simulink model "gnc_model_flightgear"  (R2026a)
settings: Solver=VariableStepAuto  StopTime=500
values from neighbouring files (symbols this model uses):
  B = [-0.25; -331.40]    [gnc_parameters.m]
  C = [-123.34, 0 ; 0, 1]    [gnc_parameters.m]
  D = [-13.51; 0]    [gnc_parameters.m]
  d2r = pi/180    (= 0.0174532925199)    [gnc_parameters.m]
  dT1 = 0.75    [gnc_parameters.m]
  dT2 = 0.25    [gnc_parameters.m]
  Elev_init = 10000    [gnc_parameters.m]
  Elev_target = 800    [gnc_parameters.m]
  Lat_init = 34.2329    [gnc_parameters.m]
  Lat_obs = 34.608485    [gnc_parameters.m]
  Lat_target = 34.6624    [gnc_parameters.m]
  Lon_init = -119.4573    [gnc_parameters.m]
  Lon_obs = -118.867712    [gnc_parameters.m]
  Lon_target = -118.7629    [gnc_parameters.m]
  m2f = 3.2811    [gnc_parameters.m]
  Vel = 3021.08    [gnc_parameters.m]
  yaw = yaw_init*d2r    [gnc_parameters.m]
undefined symbols (not defined in the file or in its folder): A, K, L
libraries: simulink x3, aerolibfltsims x2, slpidlib x1, aerolibanimutils x1
settings Model: Creator=natha  LastModifiedBy=natha

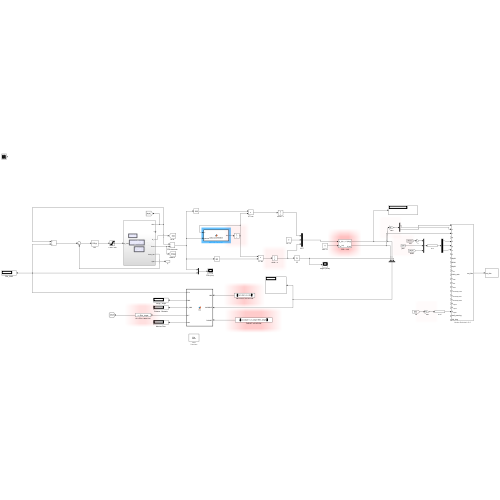
[thumbnail: Simulink's stored preview of the top-level diagram]
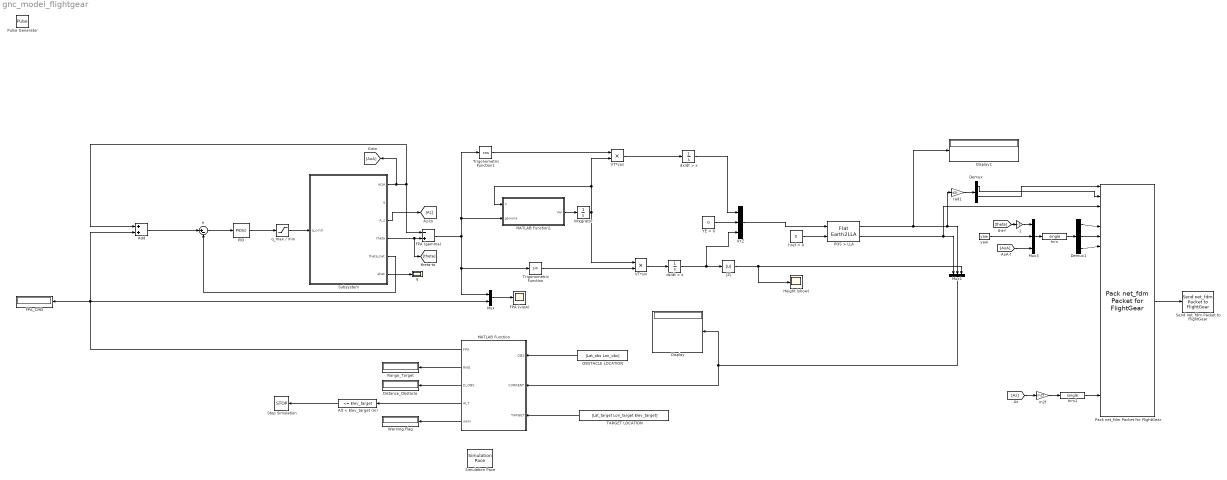
== system gnc_model_flightgear ==
  -1 : Gain  Gain=-1
  Add : Sum
  Alt < Elev_target (m) : simulink/Logic and Bit Operations/Compare To Constant  relop=<=  const=Elev_target  OutDataTypeStr=boolean
  Demux : Demux  Outputs=2
  Demux1 : Demux  Outputs=3
  Display : Display
  Display1 : Display
  Distance_Obstacle : Display
  FPA (gamma) : Sum  Inputs=-+
  FPA (view) : Scope
      settings: ActiveDisplayYMinimum=-0.063895204469408745  ActiveDisplayYMaximum=0.31656859228067386
  FPA_CMD : Display
  Height (show) : Scope
      settings: ActiveDisplayYMinimum=-1013.2400702404138  ActiveDisplayYMaximum=20440.633073900935  DataLoggingVariableName=ScopeData2
  Integrator : Integrator  InitialCondition=Vel
  MATLAB Function : MATLAB Function  TreatAsAtomicUnit=on
  MATLAB Function1 : MATLAB Function  TreatAsAtomicUnit=on
  Mux : Mux  Inputs=2
  Mux1 : Mux  Inputs=3
  Mux3 : Mux  Inputs=3
  OBSTACLE LOCATION : Constant  Value=[Lat_obs Lon_obs]
  "PID " : slpidlib/PID Controller  Controller=PID  Form=Parallel  TimeDomain=Continuous-time  UseExternalTs=off  SampleTime=-1  IntegratorMethod=Forward Euler  FilterMethod=Forward Euler  ControllerParametersSource=internal  P=-1  I=0  UseKiTs=off  D=0  UseExternalDerivativeSource=off  N=100  UseFilter=on  TunerSelectOption=Transfer Function Based (PID Tuner App)  InitialConditionSource=internal  InitialConditionForIntegrator=0  InitialConditionForFilter=0  DifferentiatorICPrevScaledInput=0  ExternalReset=none  TrackingMode=off  Kt=1  LimitOutput=off  SatLimitsSource=internal  UpperSaturationLimit=inf  LowerSaturationLimit=-inf  LinearizeAsGain=on  AntiWindupMode=none  Kb=1  LimitIntegrator=off  UpperIntegratorSaturationLimit=inf  LowerIntegratorSaturationLimit=-inf  POutMin=[]  POutMax=[]  IOutMin=[]  IOutMax=[]  DOutMin=[]  DOutMax=[]  NOutMin=[]  NOutMax=[]  SumOutMin=[]  SumOutMax=[]  SaturationOutMin=[]  SaturationOutMax=[]  PParamMin=[]  PParamMax=[]  IParamMin=[]  IParamMax=[]  DParamMin=[]  DParamMax=[]  NParamMin=[]  NParamMax=[]  KbParamMin=[]  KbParamMax=[]  KtParamMin=[]  KtParamMax=[]  KbOutMin=[]  KbOutMax=[]  KtOutMin=[]  KtOutMax=[]  IntegratorOutMin=[]  IntegratorOutMax=[]  FilterOutMin=[]  FilterOutMax=[]  SumI1OutMin=[]  SumI1OutMax=[]  SumI2OutMin=[]  SumI2OutMax=[]  SumI3OutMin=[]  SumI3OutMax=[]  SumI4OutMin=[]  SumI4OutMax=[]  SumDOutMin=[]  SumDOutMax=[]  DifferentiatorOutMin=[]  DifferentiatorOutMax=[]  FilterDiffOutCoefMin=[]  FilterDiffOutCoefMax=[]  ReciprocalOutMin=[]  ReciprocalOutMax=[]  SumDenOutMin=[]  SumDenOutMax=[]  SumNumOutMin=[]  SumNumOutMax=[]  DivideOutMin=[]  DivideOutMax=[]  UdiffTsProdOutMin=[]  UdiffTsProdOutMax=[]  NTsProdOutMin=[]  NTsProdOutMax=[]  UintegralTsProdOutMin=[]  UintegralTsProdOutMax=[]  UngainTsProdOutMin=[]  UngainTsProdOutMax=[]  ClampingZeroOutDataTypeStr=Inherit: Inherit via back propagation  ClampingZeroOutMin=[]  ClampingZeroOutMax=[]  FilterDenConstantOutDataTypeStr=Inherit: Inherit via back propagation  FilterDenConstantOutMin=[]  FilterDenConstantOutMax=[]  PCopyOutDataTypeStr=Inherit: Inherit via back propagation  PCopyOutMin=[]  PCopyOutMax=[]  NCopyOutDataTypeStr=Inherit: Inherit via back propagation  NCopyOutMin=[]  NCopyOutMax=[]  IntegratorContinuousStateAttributes=''  IntegratorStateMustResolveToSignalObject=off  IntegratorRTWStateStorageClass=Auto  FilterContinuousStateAttributes=''  FilterStateMustResolveToSignalObject=off  FilterRTWStateStorageClass=Auto  ParallelPVariant=InternalParameters  IdealPVariant=Disabled  IVariant=InternalParameters  DVariant=InternalParameters  IntegratorVariant=Continuous  SatVariant=Disabled  AWVariant=Passthrough  PCopyVariant=Disabled  TRVariant=Disabled  FdbkBlocksVariant=Forward  IdealPFdbkVariant=Disabled  SatFdbkVariant=Disabled  DerivativeFilterVariant=ContFilter  NVariant=InternalParameters  NCopyVariant=Disabled  FilterICVariant=InternalICsFilter  IntegratorICVariant=InternalICs  ExternalResetVariant=Disabled  TRSumVariant=Passthrough  SumFdbkVariant=Disabled  SumVariant=Sum_PID  TsampFilterVariant=InternalTs  TsampNgainVariant=Passthrough  TsampIntegralVariant=Disabled_SignalSpec  ExternalSaturationOutDataTypeStr=Inherit: Same as second input  DerivativeSourceVariant=ErrorSignal  PreIntVariant=InternalPreInt
  POS > LLA : FlatEarth2LLA  LL0=[Lat_init Lon_init]  psi=yaw_init
  Pack net_fdm Packet for FlightGear : aerolibfltsims/Pack net_fdm Packet for FlightGear  FlightGearVersion=v3.0  ShowPositionAttitudeInputs=on  ShowVelocityAccelerationInputs=on  ShowControlSurfacePositionInputs=off  ShowEngineFuelInputs=off  ShowLandingGearInputs=off  ShowEnvironmentInputs=off  SampleTime=1/30  packetVersion=24
  Pulse Generator : DiscretePulseGenerator  PulseType=Time based  Amplitude=0.75  Period=60  PulseWidth=50
  Range_Target : Display
  Send net_fdm Packet to FlightGear : aerolibfltsims/Send net_fdm Packet to FlightGear  DestinationIpAddress=127.0.0.1  DestinationPort=5502  LocalIpPort=-1  varLen=off  SampleTime=1/30
  Simulation Pace : aerolibanimutils/Simulation Pace  SimulationPace=2  SleepMode=Auto  OutputPaceError=off  SampleTime=1/30
  Stop Simulation : Stop
  Subsystem : Subsystem
  TARGET LOCATION : Constant  Value=[Lat_target Lon_target Elev_target]
  Trigonometric Function : Trigonometry
  Trigonometric Function1 : Trigonometry  Operator=cos
  VT*cos : Product
  VT*sin : Product
  "Warning Flag " : Display
  XYZ : Mux  Inputs=3
  YE = 0 : Constant  Value=0
  dx/dt > x : Integrator
  dz/dt > z : Integrator  InitialCondition=-Elev_init
  e : Sum  Inputs=|+-
  href = 0 : Constant  Value=0
  m2f : Gain  Gain=m2f
  q : Scope
      settings: TimeSpan=78  DataLoggingVariableName=ScopeData3  DataLoggingSaveFormat=Array
  q_max / min : Saturate
  rad1 : Gain  Gain=d2r
  to-s : DataTypeConversion  OutDataTypeStr=single  SaturateOnIntegerOverflow=off  RndMeth=Floor
  to-s1 : DataTypeConversion  OutDataTypeStr=single  SaturateOnIntegerOverflow=off  RndMeth=Floor
  yaw : Constant  Value=yaw
  |Z| : Abs  SaturateOnIntegerOverflow=off
  wires:
  Demux1/3 -> Pack net_fdm Packet for FlightGear/7
  rad1/1 -> Demux/1
  Demux1/1 -> Pack net_fdm Packet for FlightGear/5
  Demux/2 -> Pack net_fdm Packet for FlightGear/1
  [AoA] -> Mux3/3
  yaw/1 -> Mux3/2
  to-s/1 -> Demux1/1
  [theta] -> -1/1
  Mux3/1 -> to-s/1
  m2f/1 -> to-s1/1
  Demux1/2 -> Pack net_fdm Packet for FlightGear/6
  dx/dt > x/1 -> XYZ/1
  "PID "/1 -> q_max / min/1
  Subsystem/6(qhat) -> q/1
  OBSTACLE LOCATION/1 -> MATLAB Function/1(OBS)
  to-s1/1 -> Pack net_fdm Packet for FlightGear/22
  XYZ/1 -> POS > LLA/1
  Subsystem/3(A_z) -> [Az]
  |Z|/1 -> Height (show)/1, Mux1/3
  VT*cos/1 -> dx/dt > x/1
  [Az] -> m2f/1
  Mux/1 -> FPA (view)/1
  POS > LLA/1 -> Display1/1, rad1/1, Mux1/2
  Subsystem/1(AOA) -> [AoA], Add/1, FPA (gamma)/1
  POS > LLA/2 -> Pack net_fdm Packet for FlightGear/3, Mux1/1
  e/1 -> "PID "/1
  MATLAB Function/4(ALT) -> Alt < Elev_target (m)/1
  MATLAB Function/3(D_OBS) -> Distance_Obstacle/1
  Add/1 -> e/1
  q_max / min/1 -> Subsystem/1(q_cmd)
  Mux1/1 -> MATLAB Function/2(CURRENT), Display/1
  MATLAB Function/5(warn) -> "Warning Flag "/1
  MATLAB Function/2(RNG) -> Range_Target/1
  Subsystem/5(theta_hat) -> e/2
  Trigonometric Function/1 -> VT*sin/2
  dz/dt > z/1 -> XYZ/3, |Z|/1
  MATLAB Function/1(FPA) -> Add/2, FPA_CMD/1, Mux/2
  YE = 0/1 -> XYZ/2
  Alt < Elev_target (m)/1 -> Stop Simulation/1
  -1/1 -> Mux3/1
  Subsystem/4(theta) -> [theta], FPA (gamma)/2
  TARGET LOCATION/1 -> MATLAB Function/3(TARGET)
  Trigonometric Function1/1 -> VT*cos/1
  Pack net_fdm Packet for FlightGear/1 -> Send net_fdm Packet to FlightGear/1
  VT*sin/1 -> dz/dt > z/1
  Demux/1 -> Pack net_fdm Packet for FlightGear/2
  href = 0/1 -> POS > LLA/2
  FPA (gamma)/1 -> Trigonometric Function1/1, MATLAB Function1/2(gamma), Mux/1, Trigonometric Function/1
  MATLAB Function1/1(Vel) -> Integrator/1
  Integrator/1 -> VT*sin/1, VT*cos/2, MATLAB Function1/1(V)

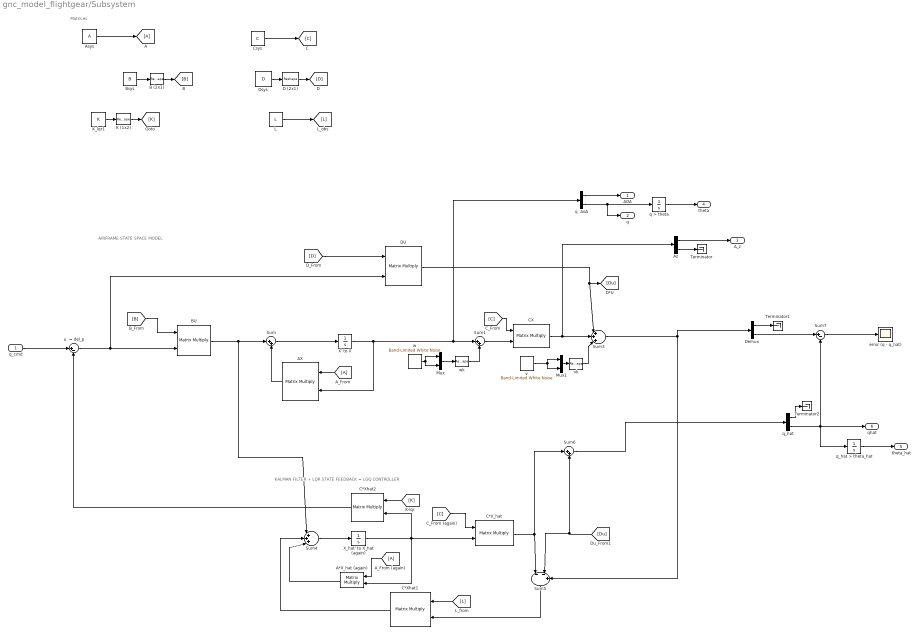
== system gnc_model_flightgear/Subsystem ==
  note: AIRFRAME STATE SPACE MODEL
  note: Matrices
  note: KALMAN FILTER + LQR STATE FEEDBACK = LGQ CONTROLLER
  q_cmd : Inport
  A : Goto
  A*X_hat (again) : Product  Multiplication=Matrix(*)
  AX : Product  Multiplication=Matrix(*)
  A_From : From
  A_From (again) : From
  Asys : Constant  Value=A
  Az : Demux  Description=Az  Outputs=2
  B (2x1) : Reshape  OutputDimensionality=Customize  OutputDimensions=[2,1]
  BU : Product  Multiplication=Matrix(*)
  Bsys : Constant  Value=B
  C*X_hat : Product  Multiplication=Matrix(*)
  C*Xhat1 : Product  Multiplication=Matrix(*)
  C*Xhat2 : Product  Multiplication=Matrix(*)
  CX : Product  Multiplication=Matrix(*)
  Csys : Constant  Value=C
  D (2x1) : Reshape  OutputDimensionality=Customize  OutputDimensions=[2,1]
  DU : Product  Multiplication=Matrix(*)
  Demux : Demux  Outputs=2
  Dsys : Constant  Value=D
  K (1x2) : Reshape  OutputDimensionality=Customize  OutputDimensions=[1,2]
  K_lqr1 : Constant  Value=K
  L : Constant  Value=L
  Mux : Mux  Inputs=2
  Mux1 : Mux  Inputs=2
  Sum : Sum  Inputs=|++
  Sum1 : Sum  Inputs=|++
  Sum3 : Sum  Inputs=|+++|
  Sum4 : Sum  Inputs=|+++|
  Sum5 : Sum  Inputs=|--+
  Sum6 : Sum  Inputs=|++
  Sum7 : Sum  Inputs=|+-
  Terminator : Terminator
  Terminator1 : Terminator
  Terminator2 : Terminator
  X' to X : Integrator
  X_hat' to X_hat (again) : Integrator
  error (q - q_hat) : Scope
  q  AoA : Demux  Outputs=2
  q > theta : Integrator
  q_hat : Demux  Outputs=2
  q_hat > theta_hat : Integrator
  u  = del_p : Sum  Inputs=|+-
  v : simulink/Sources/Band-Limited White Noise  Cov=[0.00001]  Ts=dT2  seed=[23341]
  vk : Reshape  OutputDimensionality=Customize  OutputDimensions=[2,1]
  w : simulink/Sources/Band-Limited White Noise  Cov=[0.00000001]  Ts=dT1  seed=[23341]
  wk : Reshape  OutputDimensionality=Customize  OutputDimensions=[2,1]
  AOA : Outport
  q : Outport  Port=2
  A_z : Outport  Port=3
  theta : Outport  Port=4
  theta_hat : Outport  Port=5
  qhat : Outport  Port=6
  wires:
  K_lqr1/1 -> K (1x2)/1
  X' to X/1 -> Sum1/1, q  AoA/1, AX/2
  Mux1/1 -> vk/1
  Sum6/1 -> q_hat/1
  Mux/1 -> wk/1
  q_hat/2 -> qhat/1, Sum7/2, q_hat > theta_hat/1
  Demux/2 -> Sum7/1
  Sum1/1 -> CX/2
  DU/1 -> Sum3/1, [Du]
  v/1 -> Mux1/2, Mux1/1
  Asys/1 -> A/1
  [B] -> BU/1
  wk/1 -> Sum1/2
  C*Xhat2/1 -> u  = del_p/2
  K (1x2)/1 -> [K]
  Az/2 -> Terminator/1
  L/1 -> [L]
  C*X_hat/1 -> Sum6/1, Sum5/1
  q_cmd/1 -> u  = del_p/1
  Az/1 -> A_z/1
  A_From (again)/1 -> A*X_hat (again)/1
  q_hat/1 -> Terminator2/1
  Csys/1 -> [C]
  A*X_hat (again)/1 -> Sum4/3
  Sum7/1 -> error (q - q_hat)/1
  [D] -> DU/1
  Sum4/1 -> X_hat' to X_hat (again)/1
  C*Xhat1/1 -> Sum4/2
  q > theta/1 -> theta/1
  u  = del_p/1 -> BU/2, DU/2
  w/1 -> Mux/2, Mux/1
  [C] -> CX/1
  Sum/1 -> X' to X/1
  [Du] -> Sum5/2, Sum6/2
  q  AoA/1 -> AOA/1
  q  AoA/2 -> q/1, q > theta/1
  B (2x1)/1 -> [B]
  Sum5/1 -> C*Xhat1/2
  Bsys/1 -> B (2x1)/1
  AX/1 -> Sum/2
  q_hat > theta_hat/1 -> theta_hat/1
  CX/1 -> Sum3/2, Az/1
  D (2x1)/1 -> [D]
  Sum3/1 -> Demux/1, Sum5/3
  [L] -> C*Xhat1/1
  [C] -> C*X_hat/1
  [K] -> C*Xhat2/1
  Demux/1 -> Terminator1/1
  A_From/1 -> AX/1
  Dsys/1 -> D (2x1)/1
  vk/1 -> Sum3/3
  BU/1 -> Sum/1, Sum4/1
  X_hat' to X_hat (again)/1 -> C*Xhat2/2, C*X_hat/2, A*X_hat (again)/2

== matlab function gnc_model_flightgear/MATLAB Function1 ==
  data: V input; Vel output; gamma input
function Vel = calcul_acceleration(V, gamma)
    % This parameters must be defined as "Parameters" (Workspace) dans les ports du bloc
    mass = 250; 
    g = 9.81;
    k_drag = 0.0012; % previously calculated value
    Thrust = 10000;   % Rocket booster's thrust 

    % Calcul des forces et de l'accélération
    Vel = (Thrust / mass) - (k_drag * V^2) - (g * sin(gamma));
end

== matlab function gnc_model_flightgear/MATLAB Function ==
  data: OBS input; FPA output; CURRENT input; TARGET input; RNG output; D_OBS output; ALT output; warn output
function [FPA, RNG, D_OBS, ALT, warn] = fcn(OBS, CURRENT, TARGET)
    % Earth radius in meters
    R = 6371e3 ; 
    d2r = pi/180; 

    % OBSTACLE LOCATION 
    Lat_obs = OBS(1); 
    Lon_obs = OBS(2); 
    thres = 4000; % 2500 meters threshold

    % TARGET LOCATION 
    Lat_target = TARGET(1); 
    Lon_target = TARGET(2); 
    Elev_target = TARGET(3); 

    % CURRENT LOCATION 
    Elev_cur = CURRENT(1); 
    Lat_cur = CURRENT(2); 
    Lon_cur = CURRENT(3); 

    %% distance to target 
    l1 = Lat_cur*d2r;   
    u1 = Lon_cur*d2r; 
    l2 = Lat_target*d2r; 
    u2 = Lon_target*d2r;

    dh = Elev_cur - Elev_target;  
    dl = l2 - l1 ; 
    du = u2 - u1 ; 
    a = sin(dl/2)^2 + cos(l1)*cos(l2)*sin(du/2)^2 ; 
    c = 2*atan2(sqrt(a),sqrt(1-a)) ;  
    d = R*c ; % Horizontal distance to target in meters

    %% distance from the obstacle 
    l3 = Lat_obs*d2r; 
    u3 = Lon_obs*d2r; 

    dl_obs = l3 - l1; 
    du_obs = u3 - u1; 
    a_obs = sin(dl_obs/2)^2 + cos(l1)*cos(l3)*sin(du_obs/2)^2; 
    c_obs = 2*atan2(sqrt(a_obs), sqrt(1-a_obs)); 
    d_obs = R * c_obs; % Horizontal distance to obstacle in meters

    %% current range (from target) 
    range = sqrt(d^2 + dh^2); 

    %% calculate commanded flight path setpoint based on d_obs, range 
    if d_obs >= thres         
        w = 0; 
        FPA_CMD = atan(dh/d); 
    else         
        % when in the obstacle zone, trigger warning
        w = 1; 
        FPA_CMD = -0.10; % (Around 8.5 degrees of upward slope)
    end 

    %% output variables 
    FPA = FPA_CMD; 
    RNG = range; 
    D_OBS = d_obs; 
    warn = w; 
    ALT = Elev_cur; 
end
